simulink model "NonLinear"  (R2025b)
settings: Solver=ode15s  StartTime=0.0  StopTime=100  RelTol=1e-3
PreLoadFcn:
  | Constants_and_state_space
undefined symbols (not defined in the file): CA_re, CAin_re, CB_re, QH_re, Qin_V_re, T_re, Tc_re, Tin_re
settings Model: Creator=Lenovo  LastModifiedBy=Lenovo

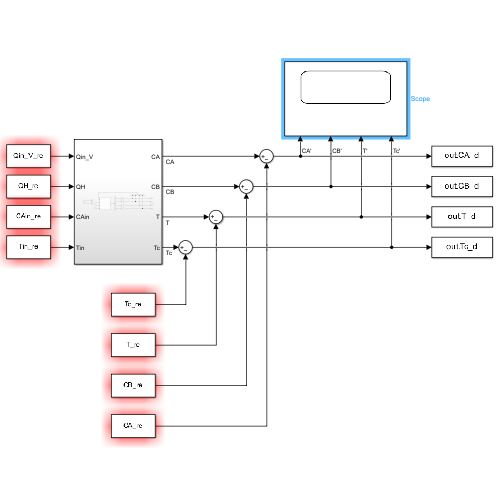
[thumbnail: Simulink's stored preview of the top-level diagram]
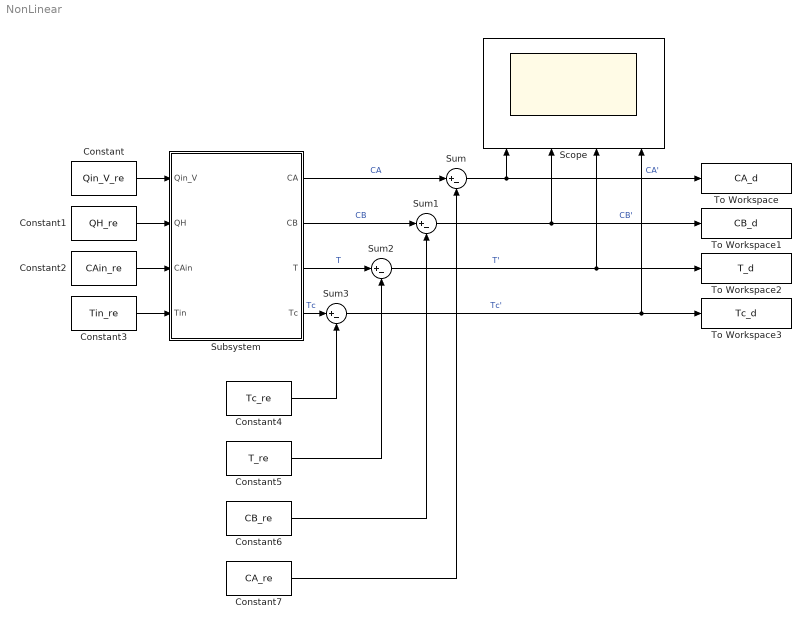
== system NonLinear ==
  Constant : Constant  Value=Qin_V_re
  Constant1 : Constant  Value=QH_re
  Constant2 : Constant  Value=CAin_re
  Constant3 : Constant  Value=Tin_re
  Constant4 : Constant  Value=Tc_re
  Constant5 : Constant  Value=T_re
  Constant6 : Constant  Value=CB_re
  Constant7 : Constant  Value=CA_re
  Scope : Scope  NumInputPorts=4
      settings: ActiveDisplayYMinimum=-2.580175396914021E-9  ActiveDisplayYMaximum=7.6367055636678217E-9
  Subsystem : Subsystem
  Sum{,1..3} (4 alike) : Sum  Inputs=|+-
  To Workspace : ToWorkspace  VariableName=CA_d  SaveFormat=Structure With Time  SampleTime=-1
  To Workspace1 : ToWorkspace  VariableName=CB_d  SaveFormat=Structure With Time  SampleTime=-1
  To Workspace2 : ToWorkspace  VariableName=T_d  SaveFormat=Structure With Time  SampleTime=-1
  To Workspace3 : ToWorkspace  VariableName=Tc_d  SaveFormat=Structure With Time  SampleTime=-1
  wires:
  Constant3/1 -> Subsystem/4(Tin)
  Constant/1 -> Subsystem/1(Qin_V)
  Constant1/1 -> Subsystem/2(QH)
  Sum/1 -> Scope/1, To Workspace/1  "CA'"
  Subsystem/1(CA) -> Sum/1  "CA"
  Sum2/1 -> To Workspace2/1, Scope/3  "T'"
  Subsystem/3(T) -> Sum2/1  "T"
  Subsystem/4(Tc) -> Sum3/1  "Tc"
  Sum3/1 -> To Workspace3/1, Scope/4  "Tc'"
  Sum1/1 -> To Workspace1/1, Scope/2  "CB'"
  Subsystem/2(CB) -> Sum1/1  "CB"
  Constant4/1 -> Sum3/2
  Constant5/1 -> Sum2/2
  Constant6/1 -> Sum1/2
  Constant7/1 -> Sum/2
  Constant2/1 -> Subsystem/3(CAin)

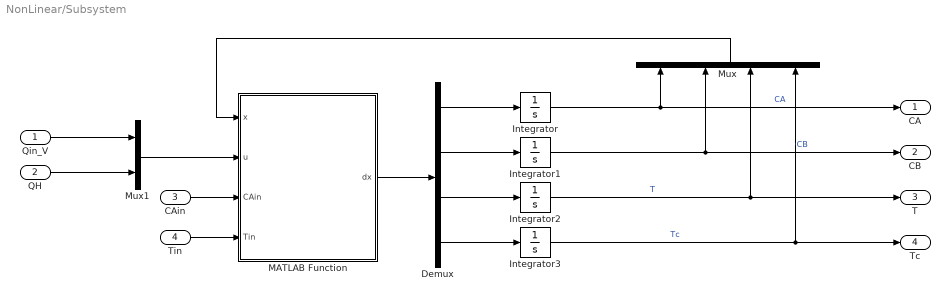
== system NonLinear/Subsystem ==
  Qin_V : Inport
  QH : Inport  Port=2
  CAin : Inport  Port=3
  Tin : Inport  Port=4
  Demux : Demux
  Integrator : Integrator  InitialCondition=CA_re
  Integrator1 : Integrator  InitialCondition=CB_re
  Integrator2 : Integrator  InitialCondition=T_re
  Integrator3 : Integrator  InitialCondition=Tc_re
  MATLAB Function : MATLAB Function  TreatAsAtomicUnit=on
  Mux : Mux
  Mux1 : Mux  Inputs=2
  CA : Outport
  CB : Outport  Port=2
  T : Outport  Port=3
  Tc : Outport  Port=4
  wires:
  Demux/3 -> Integrator2/1
  Integrator1/1 -> CB/1, Mux/2  "CB"
  Integrator/1 -> CA/1, Mux/1  "CA"
  Mux/1 -> MATLAB Function/1(x)
  Integrator2/1 -> T/1, Mux/3  "T"
  Integrator3/1 -> Tc/1, Mux/4  "Tc"
  MATLAB Function/1(dx) -> Demux/1
  Demux/2 -> Integrator1/1
  Demux/4 -> Integrator3/1
  Demux/1 -> Integrator/1
  Mux1/1 -> MATLAB Function/2(u)
  Tin/1 -> MATLAB Function/4(Tin)
  QH/1 -> Mux1/2
  CAin/1 -> MATLAB Function/3(CAin)
  Qin_V/1 -> Mux1/1

== matlab function NonLinear/Subsystem/MATLAB Function ==
  data: x input; u input; dx output; CAin input; Tin input
function dx = cstr_model(x, u, CAin, Tin)
dx = [0; 0; 0; 0]; 

% State variables

CA = x(1);
CB = x(2);
T  = x(3);
Tc = x(4);

% Manipulated variables
Qin_V = u(1);
QH    = u(2);

% Constants

V = 0.01;
Cp = 3.01;
den = 934.2; 
entAB = 4.2;
entBC = -11.0;
entAD = -41.85;
Ar = 0.215;
Kw = 4032;
mK = 5.0;
CpJ = 2.0;
k1_0 = 1.287e12;
k2_0 = 9.043e6;
E1 = -9758.3;
E2 = -8560.0;

% Arrhenius equations 

k1 = k1_0 * exp(E1 / (T + 273.15));
k2 = k2_0 * exp(E2 / (T + 273.15));

% Mass and energy balances

dx(1) = (Qin_V)*(CAin - CA) - k1*CA - k2*CA^2; % dCA/dt

dx(2) = -(Qin_V)*CB + k1*(CA - CB); %dCB/dt

dx(3) = (Qin_V)*(Tin - T) - (1/(den*Cp))*(k1*CA*entAB + k1*CB*entBC + k2*CA^2*entAD) + (Tc - T)*((Ar*Kw)/(den*Cp*V)); %dT/dt

dx(4) = (QH/(mK*CpJ)) + ((Ar*Kw)/(mK*CpJ))*(T - Tc); %dTc/dt

end
